simulink model "InductionHeating_bb_4"  (R2026b)
settings: Solver=FixedStepDiscrete  StopTime=0.008
PostLoadFcn:
  | Ts = 1e-6;Ts_fpga=10e-9;   R=3; Capa=300e-9;L=100e-6;Pejo_factor=1;
InitFcn:
  | Ts = 1e-6;Ts_fpga=10e-9;   R=3; Capa=300e-9;L=100e-6;Pejo_factor=1;
undefined symbols (not defined in the file or in its folder): DiscIntNeverNeededParam, ee_sli_rtmsupport, gcbh, isSetWhenUndefinedState, MATESOCwDio
libraries: fl_lib x67, nesl_utility x40, hdlsllib x32, simulink x15, eeGeneralControl x9, ee_lib x3
(part 3 of 7)

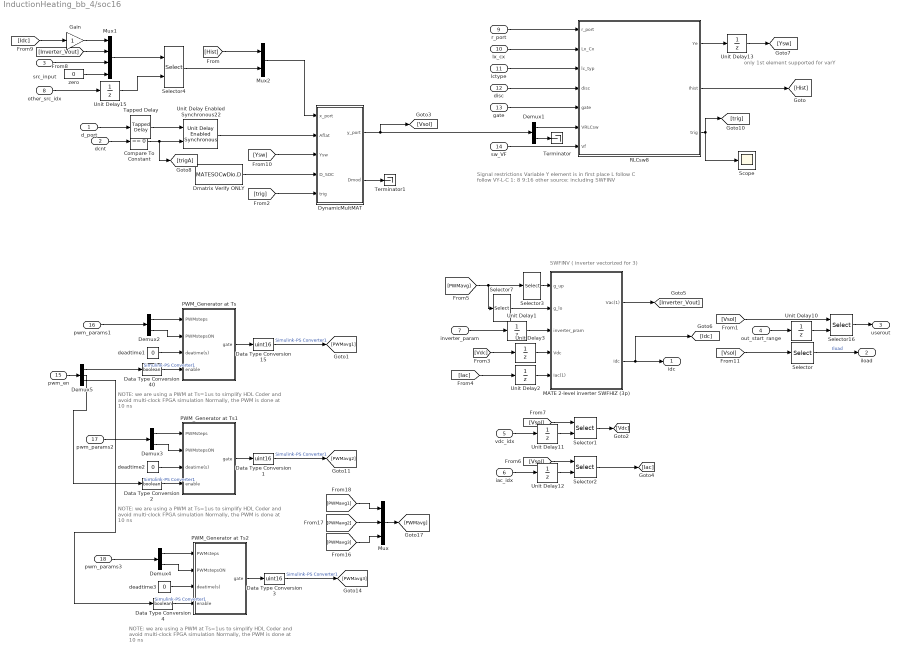
== system InductionHeating_bb_4/soc16 ==
  note: SWFINV ( inverter vectorized for 3)
  note: only 1st element supported for varY
  note: NOTE: we are using a PWM at Ts=1us to simplify HDL Coder
      | and avoid multi-clock FPGA simulation
      | Normally, the PWM is done at 10 ns
  note: Signal restrictions
      | Variable Y element is in first place
      | L follow
      | C follow
      | VY-L-C 1: 8
      | 9:16 other source: including SWFINV
  note: NOTE: we are using a PWM at Ts=1us to simplify HDL Coder
      | and avoid multi-clock FPGA simulation
      | Normally, the PWM is done at 10 ns
  note: NOTE: we are using a PWM at Ts=1us to simplify HDL Coder
      | and avoid multi-clock FPGA simulation
      | Normally, the PWM is done at 10 ns
  d_port : Inport
  dcnt : Inport  Port=2
  src_input : Inport  Port=3
  out_start_range : Inport  Port=4
  vdc_idx : Inport  Port=5
  iac_idx : Inport  Port=6
  inverter_param : Inport  Port=7
  other_src_idx : Inport  Port=8
  r_port : Inport  Port=9
  lx_cx : Inport  Port=10
  lctype : Inport  Port=11
  disc : Inport  Port=12
  gate : Inport  Port=13
  sw_VF : Inport  Port=14
  pwm_en : Inport  Port=15
  pwm_params1 : Inport  Port=16
  pwm_params2 : Inport  Port=17
  pwm_params3 : Inport  Port=18
  Compare To Constant : hdlsllib/Logic and Bit Operations/Compare To Constant  relop===  const=0  OutDataTypeStr=boolean
  Data Type Conversion1 : DataTypeConversion  OutDataTypeStr=uint16  RndMeth=Nearest  SaturateOnIntegerOverflow=off
  Data Type Conversion15 : DataTypeConversion  OutDataTypeStr=uint16  RndMeth=Nearest  SaturateOnIntegerOverflow=off
  Data Type Conversion2 : DataTypeConversion  OutDataTypeStr=boolean  RndMeth=Nearest  SaturateOnIntegerOverflow=off
  Data Type Conversion3 : DataTypeConversion  OutDataTypeStr=uint16  RndMeth=Nearest  SaturateOnIntegerOverflow=off
  Data Type Conversion4 : DataTypeConversion  OutDataTypeStr=boolean  RndMeth=Nearest  SaturateOnIntegerOverflow=off
  Data Type Conversion40 : DataTypeConversion  OutDataTypeStr=boolean  RndMeth=Nearest  SaturateOnIntegerOverflow=off
  Demux1 : Demux  Outputs=[8 8]
  Demux2 : Demux  Outputs=2
  Demux3 : Demux  Outputs=2
  Demux4 : Demux  Outputs=2
  Demux5 : Demux  Outputs=3
  Dmatrix Verify ONLY : Constant  Value=MATESOCwDio.D  OutDataTypeStr=single  SampleTime=Ts
  DynamicMultMAT : Subsystem
  Gain : Gain
  MATE 2-level inverter SWFHIZ (3p) : Subsystem  AncestorBlock=simetranss/FPGA/MATE 2-level inverter SWFHIZ (3ph)  mask(MATE Inverter Switching Function (2-level IGBT/Diode) (3-phase)){Ron=1e-3, Gpp=100, Gip=1e-6, Ts=Ts, min_charge=5}
      mask prompts: Ron "Switch Ron (Ohms)"; Gpp "Snubber resistance (Ohms)"; Gip "Snubber Capacitor (Ohms)"; Ts "Sample time (s)"; min_charge "Minimum rectifying current (A)"
      mask help:
      | This block implements a 3-phase  2-level inverter as a switching function.
      |
      | The block is Time-Step-Averaging-capable meaning that the averaging gate ON-time is averaged at each time step.
      |
      | With this approach, dead-times smaller than the sample time are accurately taken into account.
      |
      | The inverter can be in high impedance and rectifying states by selecting correctly the RC snubber.
      | Typically Rsnubber=L_load/Ts , then adjust Csnubber so Rsnubber*Csnubber=2*Ts.
      |
      | Minimum Rectifying current: In passive mode (no IGBT pulsing), this is the minimum rectifying current that is injected to the DC bus. This parameter is used to avoid unrealistic DC-bus charging when the inverter acts as a diode recfifier and do not impact in active control (gate pulsing) mode.
      |
      | The block has a constant admittance and is suitable for HDL coder.
  Mux : Mux  Inputs=3
  Mux1 : Mux  Inputs=[3 3 1 1]
  Mux2 : Mux  Inputs=[8 8]
  PWM_Generator at Ts : Subsystem
      mask Display: disp(' PWM \n Generator ')
  PWM_Generator at Ts1 : Subsystem
      mask Display: disp(' PWM \n Generator ')
  PWM_Generator at Ts2 : Subsystem
      mask Display: disp(' PWM \n Generator ')
  RLCsw8 : Subsystem  AncestorBlock=simetranss/FPGA/Variable discrete RLC  mask(Discrete variable High Accuracy Series RL or Parallel RC branch){typ=Pejovic Switch, discmeth=Backward Euler, Lon=1e-6, R=0, L=100e-6, Capa=300e-6, sbrl=on, Ts=Ts, showV=off, showI=off, Parameter11=|}
      mask Parameter11=|
      | bug list
      | Vf bug isw sign (27 08 2026)
      mask prompts: typ "Element type"; discmeth "Discretization"; Lon "Switch equivalent ON inductance (H)"; R "Initial Resistor resistance (Ohms)"; L "Initial Inductor inductance (H)"; Capa "Initial Capacitor capacitance (F)"; sbrl "Use signal-based RLC and parameter values"; Ts "Sample Time (s)"; showV "Show voltage port"; showI "Show current port"
      mask help:
      | This model implements a discretized  Series RL or Parallel RC branch that is on-line modifiable.
      |
      | On-line modifiable:  RLC parameters can be modified during simulation.
      |
      | Signals list (Vectors)
      |
      | R: resistance of either parallel RC or Series RL branch
      | Lx_Cx: inverse of capacitance (Parallel RC) or inductance (Series RL)
      | LC_type: 0 for Parallel RC, 1 for Series RL, 2 for Pejovic switch
      | disc: Choice of discretization method: 1 for Backward Euler (order 1) , 2 for Trapezoidal method (order 2), 3 for Radau IIA (5th order)
      |
      | gate: for chosen switches only, the corresponding gate signal (0 or 1)
      |
      | Use with R=0 (Series RL) to obtain a simple inductor.
      | Use with R=inf (Parallel RC) to obtain a simple capacitor.
      |
      | Note: Pejovic switches are always forced-simulated with Backward Eule with the inductance parameter value for ON state Lpejo=Ts and equivalent Open state capacitance Cpejo=Ts. Lpejo=Cpejo=Ts.
      mask init:
      | block=gcb; 
      | Xcomp=0;
      | s1=0;s2=0;s3=0;s4=0;r1=0;r2=0;l1=0;l2=0;
      | c1=0;c2=0;c3=0;c4=0;x1=0;x2=0;x3=0;x4=0;
      | 
      | MaskEnables =get_param (block ,'MaskEnables' ); 
      | discm=get_param(block,"discmeth");
      | if isequal(get_param(block,"discmeth"),'Backward Euler')
      |     dd=1;
      |     ddi=1;
      | elseif isequal(get_param(block,"discmeth"),'Trapezoidal')
      |     dd=2;
      |     ddi=2;
      | else
      |     dd=5;
      |     ddi=3;
      | end
      | sst=0;
      | br_typ=0;
      | is_sw=0;
      | 
      | % if isequal(get_param(block,"traprule"),'on')
      | %     Trapfactor=2;
      | % else
      | %     Trapfactor=1;
      | % end
      | RootMatch=0;
      | Ihist=0;
      | 
      | if isequal(get_param(block,"showV"),'on')
      |         replace_block (block ,'Followlinks' ,'on' ,'Name' ,'v' ,'BlockType' ,'Terminator' ,'Outport' ,'noprompt' ); 
      | else
      |         replace_block (block ,'Followlinks' ,'on' ,'Name' ,'v' ,'BlockType' ,'Outport' ,'Terminator' ,'noprompt' ); 
      | end
      | if isequal(get_param(block,"showI"),'on')
      |         replace_block (block ,'Followlinks' ,'on' ,'Name' ,'i' ,'BlockType' ,'Terminator' ,'Outport' ,'noprompt' ); 
      | else
      |         replace_block (block ,'Followlinks' ,'on' ,'Name' ,'i' ,'BlockType' ,'Outport' ,'Terminator' ,'noprompt' ); 
      | end
      | 
      | if isequal(get_param(block,"sbrl"),'on')
      |     replace_block (block ,'Followlinks' ,'on' ,'Name' ,'rlc' ,'BlockType' ,'Constant' ,'Inport' ,'noprompt' );
      |     MaskEnables {4 }='off' ;
      |     MaskEnables {5 }='off' ;
      |     MaskEnables {6 }='off' ;
      | else
      |     replace_block (block ,'Followlinks' ,'on' ,'Name' ,'rlc' ,'BlockType' ,'Inport' ,'Constant' ,'noprompt' );
      |     MaskEnables {4 }='on' ;
      |     MaskEnables {5 }='on' ;
      |     MaskEnables {6 }='on' ;
      | end
      | 
      | 
      | 
      | 
      | 
      | 
      | set_param (block ,'MaskEnables' ,MaskEnables ); 
      | qq='x';
      | 
      | typp=get_param(block,'typ');
      | % bp=get_param(block,'pcbp');
      | if isequal(typp,'Pejovic Switch')
      |     replace_block (block ,'Followlinks' ,'on' ,'Name' ,'gate' ,'BlockType' ,'Constant' ,'Inport' ,'noprompt' ); 
      |     %replace_block (block ,'Followlinks' ,'on' ,'Name' ,'init_in' ,'BlockType' ,'Inport' ,'Constant' ,'noprompt'  );
      |     %replace_block (block ,'Followlinks' ,'on' ,'Name' ,'init_out' ,'BlockType' ,'Outport' ,'Terminator' ,'noprompt'  );
      |     Rsw=Lon/Ts;
      |     txt='Switch';
      |     [s1,s2,s3,s4,r1,r2,l1,l2,c1,c2,c3,c4] = MATEdrawRLC('Series RLC Branch',0,1,0,'Open circuit');
      |     c2=[0 -20];
      |     c1=[30 120];
      |     qq='Switch';
      | % MaskEnables {2 }='on' ; 
      | % MaskEnables {3 }='off' ; 
      | % MaskEnables {4 }='off' ; 
      | % MaskEnables {5 }='off' ; 
      | % MaskEnables {6 }='off' ; 
      | % MaskEnables {8 }='off' ;
      | %force Backward Euler
      |     set_param(block,"discmeth",'Backward Euler')
      |     dd=1;
      |     ddi=1;
      |     is_sw=1;
      |     br_typ=0; % use Z=L/h 
      |  
      | elseif isequal(typp,'Inductor')
      |     replace_block (block ,'Followlinks' ,'on' ,'Name' ,'gate' ,'BlockType' ,'Inport' ,'Constant' ,'noprompt' ); 
      |     set_param([block '/gate'],'Value','1');
      |     replace_block (block ,'Followlinks' ,'on' ,'Name' ,'init_in' ,'BlockType' ,'Inport' ,'Constant' ,'noprompt'  ); 
      |     replace_block (block ,'Followlinks' ,'on' ,'Name' ,'init_out' ,'BlockType' ,'Outport' ,'Terminator' ,'noprompt'  );
      |  
      | 
      |     qq='Inductor';
      | % MaskEnables {2 }='off' ; 
      | % MaskEnables {3 }='on' ; 
      | % MaskEnables {4 }='off' ; 
      | % MaskEnables {5 }='on' ; 
      | % MaskEnables {6 }='off' ; 
      | % MaskEnables {8 }='off' ;
      |     x1=0;x2=0;x3=0;x4=0;
      |     if dd==5
      |         warning('Setting Inductor to Trapezoidal discretization');
      |         set_param(block,"discmeth",'Trapezoidal')
      |         dd=2;
      |     end
      |     [s1,s2,s3,s4,r1,r2,l1,l2,c1,c2,c3,c4] = MATEdrawRLC('Series RLC Branch',0,1,0,'L');
      |     [Ad,Bd1,Bd2,Cd,Dd,Y]=discRL(0,1/L,1,0,Ts,dd);
      |     Rsw=1/Y;
      | elseif isequal(typp,'Series RL')
      |     replace_block (block ,'Followlinks' ,'on' ,'Name' ,'gate' ,'BlockType' ,'Inport' ,'Constant' ,'noprompt' ); 
      |     set_param([block '/gate'],'Value','1');
      |     %replace_block (block ,'Followlinks' ,'on' ,'Name' ,'init_in' ,'BlockType' ,'Inport' ,'Constant' ,'noprompt'  ); 
      |     %replace_block (block ,'Followlinks' ,'on' ,'Name' ,'init_out' ,'BlockType' ,'Outport' ,'Terminator' ,'noprompt'  );
      | 
      |     [Ad,Bd1,Bd2,Cd,Dd,Y]=discRL(-R/L,1/L,1,0,Ts,dd);
      |     Rsw=1/Y;
      |     qq='Series RL';
      |     br_typ=0;
      |     sst=0;
      | % MaskEnables {2 }='off' ; 
      | % MaskEnables {3 }='on' ; 
      | % MaskEnables {4 }='off' ; 
      | if isequal(get_param(block,"sbrl"),'off')
      |   MaskEnables {4 }='on' ; 
      |   MaskEnables {5 }='on' ; 
      |   MaskEnables {6 }='off' ; 
      | end
      | % MaskEnables {8 }='off' ;
      |     x1=0;x2=0;x3=0;x4=0;
      |     [s1,s2,s3,s4,r1,r2,l1,l2,c1,c2,c3,c4] = MATEdrawRLC('Series RLC Branch',1,1,0,'RL');
      |     
      |     
      | elseif isequal(typp,'Parallel RC')
      |     replace_block (block ,'Followlinks' ,'on' ,'Name' ,'gate' ,'BlockType' ,'Inport' ,'Constant' ,'noprompt' ); 
      |     set_param([block '/gate'],'Value','0');
      |     %replace_block (block ,'Followlinks' ,'on' ,'Name' ,'init_in' ,'BlockType' ,'Inport' ,'Constant' ,'noprompt'  );
      |     %replace_block (block ,'Followlinks' ,'on' ,'Name' ,'init_out' ,'BlockType' ,'Outport' ,'Terminator' ,'noprompt'  );
      | if R<1e-6
      |     warndlg(['Resistance of RC block: ' block ' is very low for a Parallel RC Branch. Set R=inf if you really want an ideal capacitor with no parallel resistor.'],'MATE warning');
      | end
      |     qq='Capacitor';
      | % MaskEnables {2 }='off' ; 
      | % MaskEnables {3 }='off' ; 
      | % MaskEnables {4 }='on' ; 
      | if isequal(get_param(block,"sbrl"),'off')
      |   MaskEnables {4 }='on' ; 
      |   MaskEnables {5 }='off' ; 
      |   MaskEnables {6 }='on' ; 
      | end
      | 
      | % MaskEnables {8 }='off' ;
      |     % if dd==5 
      |     %     warning('Very low resistance. Setting Capacitor to Trapezoidal discretization');
      |     %     set_param(block,"discmeth",'Trapezoidal')
      |     %     dd=2;
      |     % end
      |     sst=1;
      |     br_typ=1;
      | 
      |     [Ad,Bd1,Bd2,Cd,Dd,Y]=discRL(-1/R/Capa,1/Capa,1,0,Ts,dd);
      |     Rsw=Y;
      | 
      |     if R>1e8
      |             [s1,s2,s3,s4,r1,r2,l1,l2,c1,c2,c3,c4,x1,x2,x3,x4] = MATEdrawRLC('Parallel RLC Branch',0,0,1,'C');
      |                 
      |     else
      |             [s1,s2,s3,s4,r1,r2,l1,l2,c1,c2,c3,c4,x1,x2,x3,x4] = MATEdrawRLC('Parallel RLC Branch',1,0,1,'RC');
      |                  s1=-20;s2=-120;s3=220;s4=120; %reframe
      | 
      |     end
      | 
      | 
      | elseif isequal(typp,'2-level inverter switch')
      |     replace_block (block ,'Followlinks' ,'on' ,'Name' ,'gate' ,'BlockType' ,'Constant' ,'Inport' ,'noprompt' ); 
      |     replace_block (block ,'Followlinks' ,'on' ,'Name' ,'init_in' ,'BlockType' ,'Constant' ,'Inport','noprompt'  );
      |     replace_block (block ,'Followlinks' ,'on' ,'Name' ,'init_out' ,'BlockType' ,'Terminator' ,'Outport' ,'noprompt'  );
      |     Rsw=Lon/Ts;
      |     txt='Inverter half';
      |     Xcomp=1;
      |     qq='Pejo Inverter Half';
      |     %force Backward Euler
      | set_param(block,'traprule','off');
      | % MaskEnables {2 }='on' ; 
      | % MaskEnables {3 }='off' ; 
      | % MaskEnables {4 }='off' ; 
      | % MaskEnables {5 }='off' ; 
      | % MaskEnables {6 }='off' ; 
      | % MaskEnables {8 }='on' ;
      |         [s1,s2,s3,s4,r1,r2,l1,l2,c1,c2,c3,c4] = MATEdrawRLC('Series RLC Branch',0,1,0,'Open circuit');
      |     c2=[0 -20];
      |     c1=[30 120];
      |         if dd==5  ||  dd==2
      |         set_param(block,"discmeth",'Backward Euler')
      |         dd=1;
      |         end
      | 
      | else
      | end
      | 
      | % if isequal(typp,'2-level inverter switch')  && isequal(bp,'on')
      | %         replace_block (block ,'Followlinks' ,'on' ,'Name' ,'Bypass' ,'BlockType' ,'Ground' ,'Inport' ,'noprompt' ); 
      | % else
      | %         replace_block (block ,'Followlinks' ,'on' ,'Name' ,'Bypass' ,'BlockType' ,'Inport' ,'Ground' ,'noprompt' ); 
      | % end
      | 
      | MaskEnables {7 }='on' ; 
      | set_param (block ,'MaskEnables' ,MaskEnables ); 
      | 
      | 
      | if Ts>2e-6
      |     %warndlg(['Sample Time of ' num2str(Ts) ' s. may be somehow large for the Pejovic switch to be accurate. Sample time below 2 us are recommended.'])
      | end
      | 
      | if isequal(get_param(block,"sbrl"),'on')
      |     x1=0;x2=0;x3=0;x4=0;
      |     [s1,s2,s3,s4,r1,r2,l1,l2,c1,c2,c3,c4] = MATEdrawRLC('Series RLC Branch',1,1,1,'RLC');
      | qq='External user choice';
      | 
      | end
      mask TypeOptions typ: Series RL | Parallel RC | Pejovic Switch
      mask TypeOptions discmeth: Backward Euler | Trapezoidal | Radau IIA 5th order
      mask DialogControl Control2 Prompt: The above RLC parameters will be used as default in SoC
      mask DialogControl Yvalue Prompt: tmp
      mask DialogControl Control4 Prompt: bugs
      mask DialogControl Control5 Prompt: Vf bug isw sign (27 08 2026)
      mask Display:
      | plot(s1,s2,s3,s4,r1,r2,l1,l2,c1,c2,c3,c4,x1,x2,x3,x4);
      | color('blue')
      | 
      | disp([qq  10 10])
  Scope : Scope
      settings: ActiveDisplayYMinimum=-0.06094  ActiveDisplayYMaximum=1.125  DataLoggingVariableName=ScopeData2
  Selector : Selector  InputPortWidth=16  IndexOptions=Index vector (dialog)  Indices=11  OutputSizes=1  RuntimeRangeChecks=off
  Selector1 : Selector  InputPortWidth=16  IndexOptions=Index vector (port)  Indices=[1:16]  OutputSizes=4  RuntimeRangeChecks=off
  Selector16 : Selector  InputPortWidth=16  IndexOptions=Starting index (port)  Indices=[1:16]  OutputSizes=5  RuntimeRangeChecks=off
  Selector2 : Selector  InputPortWidth=16  IndexOptions=Index vector (port)  Indices=[1:16]  OutputSizes=4  RuntimeRangeChecks=off
  Selector3 : Selector  InputPortWidth=6  IndexOptions=Index vector (dialog)  Indices=[1 3 5 ]  OutputSizes=1  RuntimeRangeChecks=off
  Selector4 : Selector  InputPortWidth=8  IndexOptions=Index vector (port)  Indices=[1:16]  OutputSizes=4  RuntimeRangeChecks=off
  Selector7 : Selector  InputPortWidth=6  IndexOptions=Index vector (dialog)  Indices=[1 3 5 ]+1  OutputSizes=1  RuntimeRangeChecks=off
  Tapped Delay : simulink/Discrete/Tapped Delay  vinit=0.0  samptime=-1  NumDelays=256  DelayOrder=Oldest  includeCurrent=off
      settings: LibrarySourceBlock=hdlsllib/Discrete/Tapped Delay
  Terminator : Terminator
  Terminator1 : Terminator
  Unit Delay Enabled Synchronous22 : hdlsllib/Discrete/Unit Delay Enabled Synchronous  InitialCondition=0.0  SampleTime=-1
  Unit Delay{1..3,13} (4 alike) : UnitDelay  SampleTime=Ts
  Unit Delay{10..12,15} (4 alike) : UnitDelay  InitialCondition=1  SampleTime=Ts
  deadtime1 : Constant  Value=0  SampleTime=Ts
  deadtime2 : Constant  Value=0  SampleTime=Ts
  deadtime3 : Constant  Value=0  SampleTime=Ts
  zero : Constant  Value=0  OutDataTypeStr=single  SampleTime=Ts
  idc : Outport
  iload : Outport  Port=2
  userout : Outport  Port=3
  wires:
  out_start_range/1 -> Unit Delay10/1
  Compare To Constant/1 -> [trigA], Unit Delay Enabled Synchronous22/2
  Tapped Delay/1 -> Unit Delay Enabled Synchronous22/1
  dcnt/1 -> Compare To Constant/1
  d_port/1 -> Tapped Delay/1
  [Hist] -> Mux2/1
  Unit Delay Enabled Synchronous22/1 -> DynamicMultMAT/2(Aflat)
  inverter_param/1 -> Unit Delay1/1
  Unit Delay2/1 -> MATE 2-level inverter SWFHIZ (3p)/5(Iac(1))
  [Vdc] -> Unit Delay3/1
  Unit Delay3/1 -> MATE 2-level inverter SWFHIZ (3p)/4(Vdc)
  MATE 2-level inverter SWFHIZ (3p)/2(Idc) -> [Idc], idc/1
  Selector1/1 -> [Vdc]
  [Vsol] -> Selector1/1
  [Vsol] -> Selector2/1
  Selector2/1 -> [Iac]
  [Idc] -> Gain/1
  [Inverter_Vout] -> Mux1/2
  src_input/1 -> Mux1/3
  Mux2/1 -> DynamicMultMAT/1(x_port)
  Mux1/1 -> Selector4/1
  [PWMavg] -> Selector7/1, Selector3/1
  deadtime1/1 -> PWM_Generator at Ts/3(deatime(s))
  Data Type Conversion40/1 -> PWM_Generator at Ts/4(enable)  "Simulink-PS Converter1"
  PWM_Generator at Ts/1(gate) -> Data Type Conversion15/1
  Dmatrix Verify ONLY/1 -> DynamicMultMAT/4(D_SOC)
  Demux1/1 -> RLCsw8/6(VRLCsw)
  Selector4/1 -> Mux2/2
  vdc_idx/1 -> Unit Delay11/1
  iac_idx/1 -> Unit Delay12/1
  other_src_idx/1 -> Unit Delay15/1
  zero/1 -> Mux1/4
  RLCsw8/3(trig) -> [trig], Scope/1
  RLCsw8/1(Ye) -> Unit Delay13/1
  [Ysw] -> DynamicMultMAT/3(Ysw)
  [trig] -> DynamicMultMAT/5(trig)
  MATE 2-level inverter SWFHIZ (3p)/1(Vac(1)) -> [Inverter_Vout]
  Demux1/2 -> Terminator/1
  RLCsw8/2(Ihist) -> [Hist]
  disc/1 -> RLCsw8/4(disc)
  lctype/1 -> RLCsw8/3(lc_typ)
  lx_cx/1 -> RLCsw8/2(Lx_Cx)
  r_port/1 -> RLCsw8/1(r_port)
  gate/1 -> RLCsw8/5(gate)
  Unit Delay10/1 -> Selector16/2
  pwm_params1/1 -> Demux2/1
  Unit Delay11/1 -> Selector1/2
  Unit Delay12/1 -> Selector2/2
  [Vsol] -> Selector/1
  [Vsol] -> Selector16/1
  Unit Delay15/1 -> Selector4/2
  Unit Delay13/1 -> [Ysw]
  Unit Delay1/1 -> MATE 2-level inverter SWFHIZ (3p)/3(inverter_pram)
  Data Type Conversion15/1 -> [PWMavg1]  "Simulink-PS Converter1"
  Selector/1 -> iload/1  "Iload"
  Selector3/1 -> MATE 2-level inverter SWFHIZ (3p)/1(g_up)
  Selector7/1 -> MATE 2-level inverter SWFHIZ (3p)/2(g_lo)
  Data Type Conversion1/1 -> [PWMavg2]  "Simulink-PS Converter1"
  pwm_params2/1 -> Demux3/1
  PWM_Generator at Ts1/1(gate) -> Data Type Conversion1/1
  Data Type Conversion2/1 -> PWM_Generator at Ts1/4(enable)  "Simulink-PS Converter1"
  deadtime2/1 -> PWM_Generator at Ts1/3(deatime(s))
  deadtime3/1 -> PWM_Generator at Ts2/3(deatime(s))
  Data Type Conversion4/1 -> PWM_Generator at Ts2/4(enable)  "Simulink-PS Converter1"
  PWM_Generator at Ts2/1(gate) -> Data Type Conversion3/1
  pwm_params3/1 -> Demux4/1
  Data Type Conversion3/1 -> [PWMavg3]  "Simulink-PS Converter1"
  pwm_en/1 -> Demux5/1
  Demux5/1 -> Data Type Conversion40/1
  Demux5/2 -> Data Type Conversion2/1
  Demux5/3 -> Data Type Conversion4/1
  [PWMavg2] -> Mux/2
  [PWMavg1] -> Mux/1
  [PWMavg3] -> Mux/3
  Mux/1 -> [PWMavg]
  Demux3/1 -> PWM_Generator at Ts1/1(PWMsteps)
  Demux3/2 -> PWM_Generator at Ts1/2(PWMstepsON)
  Demux4/1 -> PWM_Generator at Ts2/1(PWMsteps)
  Demux4/2 -> PWM_Generator at Ts2/2(PWMstepsON)
  Selector16/1 -> userout/1
  sw_VF/1 -> RLCsw8/7(Vf)
  Demux2/1 -> PWM_Generator at Ts/1(PWMsteps)
  Demux2/2 -> PWM_Generator at Ts/2(PWMstepsON)
  DynamicMultMAT/2(Dmod) -> Terminator1/1
  Gain/1 -> Mux1/1
  [Iac] -> Unit Delay2/1
  DynamicMultMAT/1(y_port) -> [Vsol], Demux1/1

== system InductionHeating_bb_4/Baseline Model running at 10 nanoseconds/Subsystem ==
  Current Sensor : fl_lib/Electrical/Electrical Sensors/Current Sensor
  PS-Simulink Converter : nesl_utility/PS-Simulink Converter  PhysicalDomain=network_engine_domain  SubClassName=ps_output  LeftPortType=input  RightPortType=output  PseudoPeriodic=off  Frequencies=[]  VectorFormat=1-D array  Unit=inherit  AffineConversion=off
  + : PMIOPort  Side=Left
  - : PMIOPort  Port=2  Side=Right
  i : Outport
  wires:
  PS-Simulink Converter/1 -> i/1
  connections:
  PS-Simulink Converter/LConn1 -- Current Sensor/RConn1
  Current Sensor/RConn2 -- -/RConn1
  +/RConn1 -- Current Sensor/LConn1

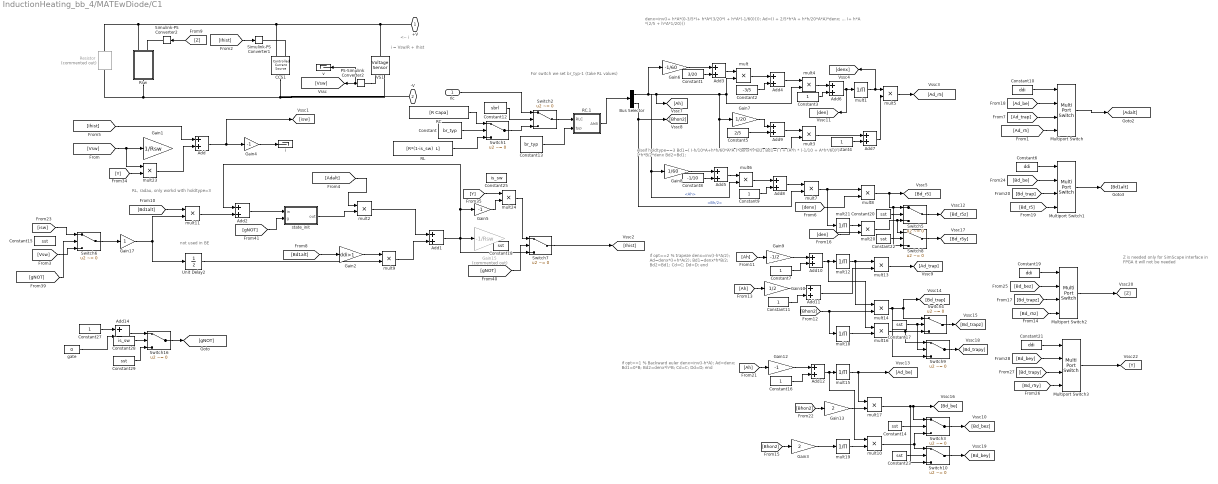
== system InductionHeating_bb_4/MATEwDiode/C1 ==
  note: not used in BE
  note: Z is needed only for SimScape interface
      | in FPGA it will not be needed
  note: i = Vsw/R + Ihist
  note: <-- i
  note: denx=inv(I+ h*A*(0-3/5*I+ h*A*(3/20*I + h*A*(-1/60))));
      | Ad=(I + 2/5*h*A + h*h/20*A*A)*denx;
      | ... I+ h*A *(2/5 + h*A*1/20)))
  note: elseif holdtype==3
      | Bd1=( I-h/10*A+h*h/60*A*A )*denx*h*B/2;
      | Bd1=( I + (A*h * (-1/10 + A*h*/60) ) )*h*B/2*denx
      | Bd2=Bd1;
  note: RL, radau, only workd with holdtype=3
  note: if opt==2 % trapeze
      | denx=inv(I-h*A/2);
      | Ad=denx*(I+h*A/2);
      | Bd1=denx*h*B/2;
      | Bd2=Bd1;
      | Cd=C;
      | Dd=D;
      | end
  note: if opt==1 % Backward euler
      | denx=inv(I-h*A);
      | Ad=denx;
      | Bd1=0*B;
      | Bd2=denx*h*B;
      | Cd=C;
      | Dd=D;
      | end
  note: For switch we set br_typ-1 (take RL values)
  rlc : Inport
  Add : Sum
  Add{1..12} (12 alike) : Sum  Inputs=2
  Add14 : Sum  Inputs=+-
  Bus Selector : BusSelector  OutputSignals=Ah,Bh/2
  CCS1 : fl_lib/Electrical/Electrical Sources/Controlled Current Source
  Constant : Constant  Value=br_typ
  Constant1 : Constant  Value=3/20  SampleTime=Ts
  Constant{6,10,19,21} (4 alike) : Constant  Value=ddi  SampleTime=Ts
  Constant{3..4,7,9,11,16,27} (7 alike) : Constant  SampleTime=Ts
  Constant12 : Constant  Value=sbrl
  Constant13 : Constant  Value=br_typ
  Constant{14..15,17..18,20,22..23,29} (8 alike) : Constant  Value=sst  SampleTime=Ts
  Constant2 : Constant  Value=-3/5  SampleTime=Ts
  Constant25 : Constant  Value=is_sw  SampleTime=Ts
  Constant28 : Constant  Value=is_sw  SampleTime=Ts
  Constant5 : Constant  Value=2/5  SampleTime=Ts
  Constant8 : Constant  Value=-1/10  SampleTime=Ts
  Gain1 : Gain  Gain=1/Rsw
  Gain10 : Gain  Gain=1/2
  Gain12 : Gain  Gain=-1
  Gain13 : Gain  Gain=2
  Gain15 : Gain  Commented=on  Gain=-1/Rsw
  Gain17 : Gain
  Gain2 : Gain  Gain=ddi>1
  Gain3 : Gain  Gain=2
  Gain4 : Gain  Gain=-1
  Gain5 : Gain  Gain=-1
  Gain6 : Gain  Gain=-1/60
  Gain7 : Gain  Gain=1/20
  Gain8 : Gain  Gain=1/60
  Gain9 : Gain  Gain=-1/2
  Multiport Switch{,1..3} (4 alike) : MultiPortSwitch  SaturateOnIntegerOverflow=off  InputSameDT=off
  PS-Simulink Converter2 : nesl_utility/PS-Simulink Converter  PhysicalDomain=network_engine_domain  SubClassName=ps_output  LeftPortType=input  RightPortType=output  PseudoPeriodic=off  Frequencies=[]  VectorFormat=inherit  Unit=inherit  AffineConversion=off
  RC : Constant  Value=[R Capa]  SampleTime=Ts
  RC.1 : Subsystem
  RL : Constant  Value="[R*(1-is_sw)  L]"  SampleTime=Ts
  Resistor : fl_lib/Electrical/Electrical Elements/Resistor  Commented=on  R=Rsw Ohm  i_specify=off  i_priority=None  i=0 A  i_nominal_specify=off  i_nominal_value=1  i_nominal_unit=A  v_specify=off  v_priority=None  v=0 V  v_nominal_specify=off  v_nominal_value=1  v_nominal_unit=V
  Rsw : Subsystem  mask(Simscape MATE variable resistance default value mask){defaultR=Rsw}
      mask prompts: defaultR "Default Resistance"
  Simulink-PS Converter1 : nesl_utility/Simulink-PS Converter  PhysicalDomain=network_engine_domain  SubClassName=ps_input  LeftPortType=input  RightPortType=output  PseudoPeriodic=off  Frequencies=[]  NoiseDistribution=none  NoiseParameters=[]  Unit=1  AffineConversion=off  FilteringAndDerivatives=provide  SimscapeFilterOrder=1  InputFilterTimeConstant=0.001  UdotUserProvided=0
  Simulink-PS Converter2 : nesl_utility/Simulink-PS Converter  PhysicalDomain=network_engine_domain  SubClassName=ps_input  LeftPortType=input  RightPortType=output  PseudoPeriodic=off  Frequencies=[]  NoiseDistribution=none  NoiseParameters=[]  Unit=1  AffineConversion=off  FilteringAndDerivatives=provide  SimscapeFilterOrder=1  InputFilterTimeConstant=0.001  UdotUserProvided=0
  Switch{1..10} (10 alike) : Switch  Criteria=u2 ~= 0  SaturateOnIntegerOverflow=off  InputSameDT=off
  Switch16 : Switch  Criteria=u2 ~= 0  Threshold=0.5  SaturateOnIntegerOverflow=off  InputSameDT=off
  Unit Delay2 : UnitDelay  SampleTime=-1
  VS1 : fl_lib/Electrical/Electrical Sensors/Voltage Sensor
  gate : Constant  Value=0
  i : Terminator
  mult{,2..11,13..14,16..17,20,23..24} (18 alike) : Product
  mult{1,12,15,18..19,21} (6 alike) : Product  Inputs=/
  state_init : Subsystem
  v : Terminator
  +V : PMIOPort  Side=Left
  -V : PMIOPort  Port=2  Side=Right
  wires:
  Switch7/1 -> [Ihist]
  gate/1 -> Add14/2
  mult20/1 -> Switch8/1, Switch5/3
  Constant20/1 -> Switch5/2
  Switch5/1 -> [Bd_r5z]
  mult21/1 -> mult20/1
  [den] -> mult20/2
  Switch3/1 -> [Bd_bez]
  Constant14/1 -> Switch3/2
  mult17/1 -> Switch10/3, [Bd_be], Switch3/1
  mult10/1 -> Switch10/1, Switch3/3
  mult19/1 -> mult10/2
  [Bhon2] -> Gain3/1
  Gain3/1 -> mult19/1
  mult18/1 -> mult16/2
  Constant13/1 -> RC.1/2(typ)
  RC.1/1(AhB) -> Bus Selector/1
  Constant12/1 -> Switch2/2
  rlc/1 -> Switch2/1
  Switch2/1 -> RC.1/1(RLC)
  Switch1/1 -> Switch2/3
  Constant/1 -> Switch1/2
  RL/1 -> Switch1/3
  RC/1 -> Switch1/1
  Gain2/1 -> mult9/1
  Constant10/1 -> Multiport Switch/1
  Constant6/1 -> Multiport Switch1/1
  Multiport Switch1/1 -> [Bd1alt]
  [Bd_be] -> Multiport Switch1/2
  [Bd_trap] -> Multiport Switch1/3
  [Bd_r5] -> Multiport Switch1/4
  Multiport Switch/1 -> [Adalt]
  [Ad_be] -> Multiport Switch/2
  [Ad_trap] -> Multiport Switch/3
  [Ad_r5] -> Multiport Switch/4
  Gain13/1 -> mult17/2
  [Ah] -> Gain12/1
  Gain12/1 -> Add12/1
  Constant16/1 -> Add12/2
  Add12/1 -> mult15/1, mult10/1
  [Bhon2] -> Gain13/1
  mult15/1 -> mult17/1, [Ad_be]
  mult11/1 -> Add2/2
  [Bd1alt] -> mult11/1
  [Bd1alt] -> Gain2/1
  mult9/1 -> Add1/2
  mult13/1 -> [Ad_trap]
  [Bhon2] -> mult14/2, mult18/1
  mult12/1 -> mult13/1, mult14/1
  [Ah] -> Gain10/1
  Gain10/1 -> Add11/1
  Constant11/1 -> Add11/2
  Add11/1 -> mult13/2
  Add10/1 -> mult12/1, mult16/1
  Constant7/1 -> Add10/2
  Gain9/1 -> Add10/1
  [Ah] -> Gain9/1
  [Z] -> Simulink-PS Converter2/1
  Bus Selector/2 -> [Bhon2], mult7/2  "<Bh/2>"
  Bus Selector/1 -> mult6/2, Gain8/1, mult/2, mult4/2, Gain7/1, mult3/2, [Ah], Gain6/1  "<Ah>"
  [denx] -> mult8/2
  mult7/1 -> mult8/1, mult21/1
  Add8/1 -> mult7/1
  Gain8/1 -> Add5/1
  Constant8/1 -> Add5/2
  mult6/1 -> Add8/1
  Add5/1 -> mult6/1
  Constant9/1 -> Add8/2
  mult5/1 -> [Ad_r5]
  mult1/1 -> mult5/1, [denx]
  [Adalt] -> mult2/1
  Add7/1 -> mult5/2
  mult3/1 -> Add7/1
  Gain7/1 -> Add9/1
  Add9/1 -> mult3/1
  Constant5/1 -> Add9/2
  Constant4/1 -> Add7/2
  Add6/1 -> mult1/1, [den]
  Constant3/1 -> Add6/2
  mult4/1 -> Add6/1
  Add4/1 -> mult4/1
  Constant2/1 -> Add4/2
  Add3/1 -> mult/1
  mult/1 -> Add4/1
  Constant1/1 -> Add3/2
  Gain6/1 -> Add3/1
  Unit Delay2/1 -> mult9/2
  Add1/1 -> Switch7/3, Gain5/1, Add2/1, Gain15/1
  Add2/1 -> state_init/1(in)
  Gain4/1 -> i/1
  [Ihist] -> Add/1
  PS-Simulink Converter2/1 -> [Vsw], v/1
  [Vsw] -> mult23/1, Gain1/1
  [Ihist] -> Simulink-PS Converter1/1
  Add/1 -> [isw], Gain4/1
  Switch6/1 -> Gain17/1
  [Vsw] -> Switch6/3
  [isw] -> Switch6/1
  mult2/1 -> Add1/1
  [Bd_r5z] -> Multiport Switch2/4
  [Bd_trapz] -> Multiport Switch2/3
  [Bd_bez] -> Multiport Switch2/2
  Multiport Switch2/1 -> [Z]
  Constant19/1 -> Multiport Switch2/1
  mult8/1 -> [Bd_r5], Switch8/3, Switch5/1
  Switch4/1 -> [Bd_trapz]
  Constant21/1 -> Multiport Switch3/1
  [Bd_bey] -> Multiport Switch3/2
  [Bd_trapy] -> Multiport Switch3/3
  [Bd_r5y] -> Multiport Switch3/4
  Switch8/1 -> [Bd_r5y]
  Constant22/1 -> Switch8/2
  Switch9/1 -> [Bd_trapy]
  Constant17/1 -> Switch9/2, Switch4/2
  mult16/1 -> Switch9/1, Switch4/3
  mult14/1 -> Switch9/3, [Bd_trap], Switch4/1
  Switch10/1 -> [Bd_bey]
  Constant23/1 -> Switch10/2
  Multiport Switch3/1 -> [Y]
  [Y] -> mult23/2
  mult23/1 -> Add/2
  mult24/1 -> Switch7/1
  [Y] -> mult24/1
  Gain5/1 -> mult24/2
  Gain17/1 -> mult11/2, Unit Delay2/1
  Constant27/1 -> Add14/1
  [gNOT] -> Switch6/2
  [gNOT] -> Switch7/2
  state_init/1(out) -> mult2/2
  [gNOT] -> state_init/2(g)
  Add14/1 -> Switch16/1
  Switch16/1 -> [gNOT]
  Constant28/1 -> Switch16/2
  Constant29/1 -> Switch16/3
  connections:
  Simulink-PS Converter2/RConn1 -- Rsw/LConn2
  Rsw/RConn1 -- Resistor/RConn1 -- VS1/RConn2 -- -V/RConn1 -- CCS1/LConn1
  PS-Simulink Converter2/LConn1 -- VS1/RConn1
  CCS1/RConn1 -- Simulink-PS Converter1/RConn1
  Rsw/LConn1 -- Resistor/LConn1 -- VS1/LConn1 -- +V/RConn1 -- CCS1/RConn2

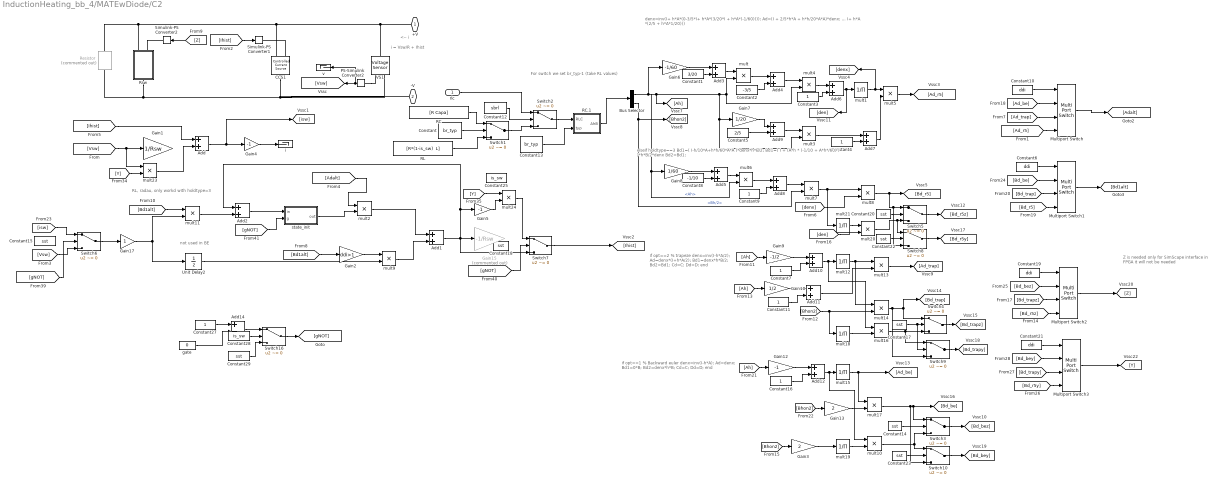
== system InductionHeating_bb_4/MATEwDiode/C2 ==
  note: not used in BE
  note: Z is needed only for SimScape interface
      | in FPGA it will not be needed
  note: i = Vsw/R + Ihist
  note: <-- i
  note: denx=inv(I+ h*A*(0-3/5*I+ h*A*(3/20*I + h*A*(-1/60))));
      | Ad=(I + 2/5*h*A + h*h/20*A*A)*denx;
      | ... I+ h*A *(2/5 + h*A*1/20)))
  note: elseif holdtype==3
      | Bd1=( I-h/10*A+h*h/60*A*A )*denx*h*B/2;
      | Bd1=( I + (A*h * (-1/10 + A*h*/60) ) )*h*B/2*denx
      | Bd2=Bd1;
  note: RL, radau, only workd with holdtype=3
  note: if opt==2 % trapeze
      | denx=inv(I-h*A/2);
      | Ad=denx*(I+h*A/2);
      | Bd1=denx*h*B/2;
      | Bd2=Bd1;
      | Cd=C;
      | Dd=D;
      | end
  note: if opt==1 % Backward euler
      | denx=inv(I-h*A);
      | Ad=denx;
      | Bd1=0*B;
      | Bd2=denx*h*B;
      | Cd=C;
      | Dd=D;
      | end
  note: For switch we set br_typ-1 (take RL values)
  rlc : Inport
  Add : Sum
  Add{1..12} (12 alike) : Sum  Inputs=2
  Add14 : Sum  Inputs=+-
  Bus Selector : BusSelector  OutputSignals=Ah,Bh/2
  CCS1 : fl_lib/Electrical/Electrical Sources/Controlled Current Source
  Constant : Constant  Value=br_typ
  Constant1 : Constant  Value=3/20  SampleTime=Ts
  Constant{6,10,19,21} (4 alike) : Constant  Value=ddi  SampleTime=Ts
  Constant{3..4,7,9,11,16,27} (7 alike) : Constant  SampleTime=Ts
  Constant12 : Constant  Value=sbrl
  Constant13 : Constant  Value=br_typ
  Constant{14..15,17..18,20,22..23,29} (8 alike) : Constant  Value=sst  SampleTime=Ts
  Constant2 : Constant  Value=-3/5  SampleTime=Ts
  Constant25 : Constant  Value=is_sw  SampleTime=Ts
  Constant28 : Constant  Value=is_sw  SampleTime=Ts
  Constant5 : Constant  Value=2/5  SampleTime=Ts
  Constant8 : Constant  Value=-1/10  SampleTime=Ts
  Gain1 : Gain  Gain=1/Rsw
  Gain10 : Gain  Gain=1/2
  Gain12 : Gain  Gain=-1
  Gain13 : Gain  Gain=2
  Gain15 : Gain  Commented=on  Gain=-1/Rsw
  Gain17 : Gain
  Gain2 : Gain  Gain=ddi>1
  Gain3 : Gain  Gain=2
  Gain4 : Gain  Gain=-1
  Gain5 : Gain  Gain=-1
  Gain6 : Gain  Gain=-1/60
  Gain7 : Gain  Gain=1/20
  Gain8 : Gain  Gain=1/60
  Gain9 : Gain  Gain=-1/2
  Multiport Switch{,1..3} (4 alike) : MultiPortSwitch  SaturateOnIntegerOverflow=off  InputSameDT=off
  PS-Simulink Converter2 : nesl_utility/PS-Simulink Converter  PhysicalDomain=network_engine_domain  SubClassName=ps_output  LeftPortType=input  RightPortType=output  PseudoPeriodic=off  Frequencies=[]  VectorFormat=inherit  Unit=inherit  AffineConversion=off
  RC : Constant  Value=[R Capa]  SampleTime=Ts
  RC.1 : Subsystem
  RL : Constant  Value="[R*(1-is_sw)  L]"  SampleTime=Ts
  Resistor : fl_lib/Electrical/Electrical Elements/Resistor  Commented=on  R=Rsw Ohm  i_specify=off  i_priority=None  i=0 A  i_nominal_specify=off  i_nominal_value=1  i_nominal_unit=A  v_specify=off  v_priority=None  v=0 V  v_nominal_specify=off  v_nominal_value=1  v_nominal_unit=V
  Rsw : Subsystem  mask(Simscape MATE variable resistance default value mask){defaultR=Rsw}
      mask prompts: defaultR "Default Resistance"
  Simulink-PS Converter1 : nesl_utility/Simulink-PS Converter  PhysicalDomain=network_engine_domain  SubClassName=ps_input  LeftPortType=input  RightPortType=output  PseudoPeriodic=off  Frequencies=[]  NoiseDistribution=none  NoiseParameters=[]  Unit=1  AffineConversion=off  FilteringAndDerivatives=provide  SimscapeFilterOrder=1  InputFilterTimeConstant=0.001  UdotUserProvided=0
  Simulink-PS Converter2 : nesl_utility/Simulink-PS Converter  PhysicalDomain=network_engine_domain  SubClassName=ps_input  LeftPortType=input  RightPortType=output  PseudoPeriodic=off  Frequencies=[]  NoiseDistribution=none  NoiseParameters=[]  Unit=1  AffineConversion=off  FilteringAndDerivatives=provide  SimscapeFilterOrder=1  InputFilterTimeConstant=0.001  UdotUserProvided=0
  Switch{1..10} (10 alike) : Switch  Criteria=u2 ~= 0  SaturateOnIntegerOverflow=off  InputSameDT=off
  Switch16 : Switch  Criteria=u2 ~= 0  Threshold=0.5  SaturateOnIntegerOverflow=off  InputSameDT=off
  Unit Delay2 : UnitDelay  SampleTime=-1
  VS1 : fl_lib/Electrical/Electrical Sensors/Voltage Sensor
  gate : Constant  Value=0
  i : Terminator
  mult{,2..11,13..14,16..17,20,23..24} (18 alike) : Product
  mult{1,12,15,18..19,21} (6 alike) : Product  Inputs=/
  state_init : Subsystem
  v : Terminator
  +V : PMIOPort  Side=Left
  -V : PMIOPort  Port=2  Side=Right
  wires:
  Switch7/1 -> [Ihist]
  gate/1 -> Add14/2
  mult20/1 -> Switch8/1, Switch5/3
  Constant20/1 -> Switch5/2
  Switch5/1 -> [Bd_r5z]
  mult21/1 -> mult20/1
  [den] -> mult20/2
  Switch3/1 -> [Bd_bez]
  Constant14/1 -> Switch3/2
  mult17/1 -> Switch10/3, [Bd_be], Switch3/1
  mult10/1 -> Switch10/1, Switch3/3
  mult19/1 -> mult10/2
  [Bhon2] -> Gain3/1
  Gain3/1 -> mult19/1
  mult18/1 -> mult16/2
  Constant13/1 -> RC.1/2(typ)
  RC.1/1(AhB) -> Bus Selector/1
  Constant12/1 -> Switch2/2
  rlc/1 -> Switch2/1
  Switch2/1 -> RC.1/1(RLC)
  Switch1/1 -> Switch2/3
  Constant/1 -> Switch1/2
  RL/1 -> Switch1/3
  RC/1 -> Switch1/1
  Gain2/1 -> mult9/1
  Constant10/1 -> Multiport Switch/1
  Constant6/1 -> Multiport Switch1/1
  Multiport Switch1/1 -> [Bd1alt]
  [Bd_be] -> Multiport Switch1/2
  [Bd_trap] -> Multiport Switch1/3
  [Bd_r5] -> Multiport Switch1/4
  Multiport Switch/1 -> [Adalt]
  [Ad_be] -> Multiport Switch/2
  [Ad_trap] -> Multiport Switch/3
  [Ad_r5] -> Multiport Switch/4
  Gain13/1 -> mult17/2
  [Ah] -> Gain12/1
  Gain12/1 -> Add12/1
  Constant16/1 -> Add12/2
  Add12/1 -> mult15/1, mult10/1
  [Bhon2] -> Gain13/1
  mult15/1 -> mult17/1, [Ad_be]
  mult11/1 -> Add2/2
  [Bd1alt] -> mult11/1
  [Bd1alt] -> Gain2/1
  mult9/1 -> Add1/2
  mult13/1 -> [Ad_trap]
  [Bhon2] -> mult14/2, mult18/1
  mult12/1 -> mult13/1, mult14/1
  [Ah] -> Gain10/1
  Gain10/1 -> Add11/1
  Constant11/1 -> Add11/2
  Add11/1 -> mult13/2
  Add10/1 -> mult12/1, mult16/1
  Constant7/1 -> Add10/2
  Gain9/1 -> Add10/1
  [Ah] -> Gain9/1
  [Z] -> Simulink-PS Converter2/1
  Bus Selector/2 -> [Bhon2], mult7/2  "<Bh/2>"
  Bus Selector/1 -> mult6/2, Gain8/1, mult/2, mult4/2, Gain7/1, mult3/2, [Ah], Gain6/1  "<Ah>"
  [denx] -> mult8/2
  mult7/1 -> mult8/1, mult21/1
  Add8/1 -> mult7/1
  Gain8/1 -> Add5/1
  Constant8/1 -> Add5/2
  mult6/1 -> Add8/1
  Add5/1 -> mult6/1
  Constant9/1 -> Add8/2
  mult5/1 -> [Ad_r5]
  mult1/1 -> mult5/1, [denx]
  [Adalt] -> mult2/1
  Add7/1 -> mult5/2
  mult3/1 -> Add7/1
  Gain7/1 -> Add9/1
  Add9/1 -> mult3/1
  Constant5/1 -> Add9/2
  Constant4/1 -> Add7/2
  Add6/1 -> mult1/1, [den]
  Constant3/1 -> Add6/2
  mult4/1 -> Add6/1
  Add4/1 -> mult4/1
  Constant2/1 -> Add4/2
  Add3/1 -> mult/1
  mult/1 -> Add4/1
  Constant1/1 -> Add3/2
  Gain6/1 -> Add3/1
  Unit Delay2/1 -> mult9/2
  Add1/1 -> Switch7/3, Gain5/1, Add2/1, Gain15/1
  Add2/1 -> state_init/1(in)
  Gain4/1 -> i/1
  [Ihist] -> Add/1
  PS-Simulink Converter2/1 -> [Vsw], v/1
  [Vsw] -> mult23/1, Gain1/1
  [Ihist] -> Simulink-PS Converter1/1
  Add/1 -> [isw], Gain4/1
  Switch6/1 -> Gain17/1
  [Vsw] -> Switch6/3
  [isw] -> Switch6/1
  mult2/1 -> Add1/1
  [Bd_r5z] -> Multiport Switch2/4
  [Bd_trapz] -> Multiport Switch2/3
  [Bd_bez] -> Multiport Switch2/2
  Multiport Switch2/1 -> [Z]
  Constant19/1 -> Multiport Switch2/1
  mult8/1 -> [Bd_r5], Switch8/3, Switch5/1
  Switch4/1 -> [Bd_trapz]
  Constant21/1 -> Multiport Switch3/1
  [Bd_bey] -> Multiport Switch3/2
  [Bd_trapy] -> Multiport Switch3/3
  [Bd_r5y] -> Multiport Switch3/4
  Switch8/1 -> [Bd_r5y]
  Constant22/1 -> Switch8/2
  Switch9/1 -> [Bd_trapy]
  Constant17/1 -> Switch9/2, Switch4/2
  mult16/1 -> Switch9/1, Switch4/3
  mult14/1 -> Switch9/3, [Bd_trap], Switch4/1
  Switch10/1 -> [Bd_bey]
  Constant23/1 -> Switch10/2
  Multiport Switch3/1 -> [Y]
  [Y] -> mult23/2
  mult23/1 -> Add/2
  mult24/1 -> Switch7/1
  [Y] -> mult24/1
  Gain5/1 -> mult24/2
  Gain17/1 -> mult11/2, Unit Delay2/1
  Constant27/1 -> Add14/1
  [gNOT] -> Switch6/2
  [gNOT] -> Switch7/2
  state_init/1(out) -> mult2/2
  [gNOT] -> state_init/2(g)
  Add14/1 -> Switch16/1
  Switch16/1 -> [gNOT]
  Constant28/1 -> Switch16/2
  Constant29/1 -> Switch16/3
  connections:
  Simulink-PS Converter2/RConn1 -- Rsw/LConn2
  Rsw/RConn1 -- Resistor/RConn1 -- VS1/RConn2 -- -V/RConn1 -- CCS1/LConn1
  PS-Simulink Converter2/LConn1 -- VS1/RConn1
  CCS1/RConn1 -- Simulink-PS Converter1/RConn1
  Rsw/LConn1 -- Resistor/LConn1 -- VS1/LConn1 -- +V/RConn1 -- CCS1/RConn2

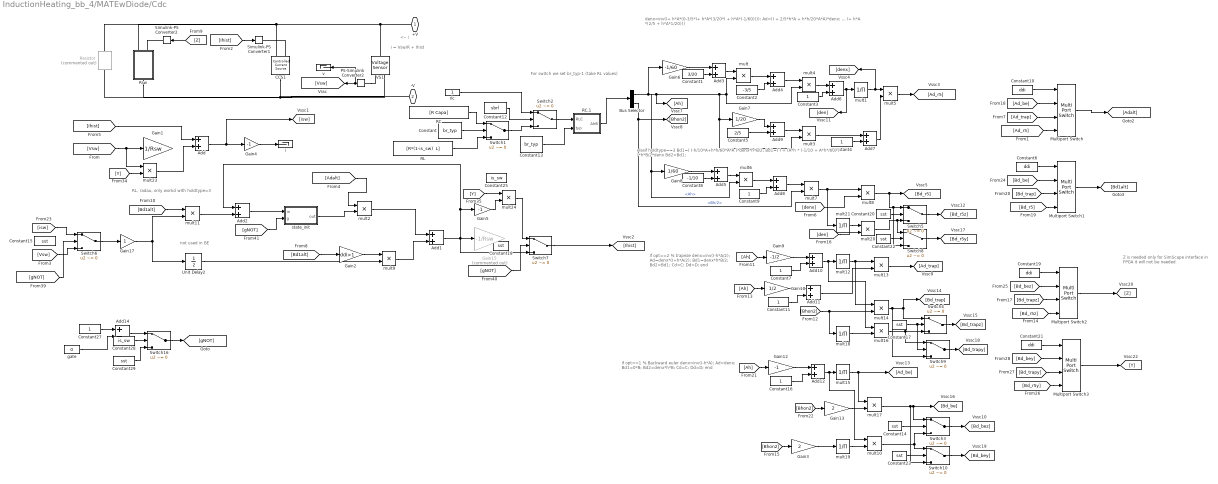
== system InductionHeating_bb_4/MATEwDiode/Cdc ==
  note: For switch we set br_typ-1 (take RL values)
  note: if opt==1 % Backward euler
      | denx=inv(I-h*A);
      | Ad=denx;
      | Bd1=0*B;
      | Bd2=denx*h*B;
      | Cd=C;
      | Dd=D;
      | end
  note: if opt==2 % trapeze
      | denx=inv(I-h*A/2);
      | Ad=denx*(I+h*A/2);
      | Bd1=denx*h*B/2;
      | Bd2=Bd1;
      | Cd=C;
      | Dd=D;
      | end
  note: RL, radau, only workd with holdtype=3
  note: elseif holdtype==3
      | Bd1=( I-h/10*A+h*h/60*A*A )*denx*h*B/2;
      | Bd1=( I + (A*h * (-1/10 + A*h*/60) ) )*h*B/2*denx
      | Bd2=Bd1;
  note: denx=inv(I+ h*A*(0-3/5*I+ h*A*(3/20*I + h*A*(-1/60))));
      | Ad=(I + 2/5*h*A + h*h/20*A*A)*denx;
      | ... I+ h*A *(2/5 + h*A*1/20)))
  note: <-- i
  note: i = Vsw/R + Ihist
  note: Z is needed only for SimScape interface
      | in FPGA it will not be needed
  note: not used in BE
  Add : Sum
  Add{1..12} (12 alike) : Sum  Inputs=2
  Add14 : Sum  Inputs=+-
  Bus Selector : BusSelector  OutputSignals=Ah,Bh/2
  CCS1 : fl_lib/Electrical/Electrical Sources/Controlled Current Source
  Constant : Constant  Value=br_typ
  Constant1 : Constant  Value=3/20  SampleTime=Ts
  Constant{6,10,19,21} (4 alike) : Constant  Value=ddi  SampleTime=Ts
  Constant{3..4,7,9,11,16,27} (7 alike) : Constant  SampleTime=Ts
  Constant12 : Constant  Value=sbrl
  Constant13 : Constant  Value=br_typ
  Constant{14..15,17..18,20,22..23,29} (8 alike) : Constant  Value=sst  SampleTime=Ts
  Constant2 : Constant  Value=-3/5  SampleTime=Ts
  Constant25 : Constant  Value=is_sw  SampleTime=Ts
  Constant28 : Constant  Value=is_sw  SampleTime=Ts
  Constant5 : Constant  Value=2/5  SampleTime=Ts
  Constant8 : Constant  Value=-1/10  SampleTime=Ts
  Gain1 : Gain  Gain=1/Rsw
  Gain10 : Gain  Gain=1/2
  Gain12 : Gain  Gain=-1
  Gain13 : Gain  Gain=2
  Gain15 : Gain  Commented=on  Gain=-1/Rsw
  Gain17 : Gain
  Gain2 : Gain  Gain=ddi>1
  Gain3 : Gain  Gain=2
  Gain4 : Gain  Gain=-1
  Gain5 : Gain  Gain=-1
  Gain6 : Gain  Gain=-1/60
  Gain7 : Gain  Gain=1/20
  Gain8 : Gain  Gain=1/60
  Gain9 : Gain  Gain=-1/2
  Multiport Switch{,1..3} (4 alike) : MultiPortSwitch  SaturateOnIntegerOverflow=off  InputSameDT=off
  PS-Simulink Converter2 : nesl_utility/PS-Simulink Converter  PhysicalDomain=network_engine_domain  SubClassName=ps_output  LeftPortType=input  RightPortType=output  PseudoPeriodic=off  Frequencies=[]  VectorFormat=inherit  Unit=inherit  AffineConversion=off
  RC : Constant  Value=[R Capa]  SampleTime=Ts
  RC.1 : Subsystem
  RL : Constant  Value="[R*(1-is_sw)  L]"  SampleTime=Ts
  Resistor : fl_lib/Electrical/Electrical Elements/Resistor  Commented=on  R=Rsw Ohm  i_specify=off  i_priority=None  i=0 A  i_nominal_specify=off  i_nominal_value=1  i_nominal_unit=A  v_specify=off  v_priority=None  v=0 V  v_nominal_specify=off  v_nominal_value=1  v_nominal_unit=V
  Rsw : Subsystem  mask(Simscape MATE variable resistance default value mask){defaultR=Rsw}
      mask prompts: defaultR "Default Resistance"
  Simulink-PS Converter1 : nesl_utility/Simulink-PS Converter  PhysicalDomain=network_engine_domain  SubClassName=ps_input  LeftPortType=input  RightPortType=output  PseudoPeriodic=off  Frequencies=[]  NoiseDistribution=none  NoiseParameters=[]  Unit=1  AffineConversion=off  FilteringAndDerivatives=provide  SimscapeFilterOrder=1  InputFilterTimeConstant=0.001  UdotUserProvided=0
  Simulink-PS Converter2 : nesl_utility/Simulink-PS Converter  PhysicalDomain=network_engine_domain  SubClassName=ps_input  LeftPortType=input  RightPortType=output  PseudoPeriodic=off  Frequencies=[]  NoiseDistribution=none  NoiseParameters=[]  Unit=1  AffineConversion=off  FilteringAndDerivatives=provide  SimscapeFilterOrder=1  InputFilterTimeConstant=0.001  UdotUserProvided=0
  Switch{1..10} (10 alike) : Switch  Criteria=u2 ~= 0  SaturateOnIntegerOverflow=off  InputSameDT=off
  Switch16 : Switch  Criteria=u2 ~= 0  Threshold=0.5  SaturateOnIntegerOverflow=off  InputSameDT=off
  Unit Delay2 : UnitDelay  SampleTime=-1
  VS1 : fl_lib/Electrical/Electrical Sensors/Voltage Sensor
  gate : Constant  Value=0
  i : Terminator
  mult{,2..11,13..14,16..17,20,23..24} (18 alike) : Product
  mult{1,12,15,18..19,21} (6 alike) : Product  Inputs=/
  rlc : Constant
  state_init : Subsystem
  v : Terminator
  +V : PMIOPort  Side=Left
  -V : PMIOPort  Port=2  Side=Right
  wires:
  Constant29/1 -> Switch16/3
  Constant28/1 -> Switch16/2
  Switch16/1 -> [gNOT]
  Add14/1 -> Switch16/1
  [gNOT] -> state_init/2(g)
  state_init/1(out) -> mult2/2
  [gNOT] -> Switch7/2
  [gNOT] -> Switch6/2
  Constant27/1 -> Add14/1
  Gain17/1 -> Unit Delay2/1, mult11/2
  Gain5/1 -> mult24/2
  [Y] -> mult24/1
  mult24/1 -> Switch7/1
  mult23/1 -> Add/2
  [Y] -> mult23/2
  Multiport Switch3/1 -> [Y]
  Constant23/1 -> Switch10/2
  Switch10/1 -> [Bd_bey]
  mult14/1 -> Switch4/1, [Bd_trap], Switch9/3
  mult16/1 -> Switch4/3, Switch9/1
  Constant17/1 -> Switch4/2, Switch9/2
  Switch9/1 -> [Bd_trapy]
  Constant22/1 -> Switch8/2
  Switch8/1 -> [Bd_r5y]
  [Bd_r5y] -> Multiport Switch3/4
  [Bd_trapy] -> Multiport Switch3/3
  [Bd_bey] -> Multiport Switch3/2
  Constant21/1 -> Multiport Switch3/1
  Switch4/1 -> [Bd_trapz]
  mult8/1 -> Switch5/1, Switch8/3, [Bd_r5]
  Constant19/1 -> Multiport Switch2/1
  Multiport Switch2/1 -> [Z]
  [Bd_bez] -> Multiport Switch2/2
  [Bd_trapz] -> Multiport Switch2/3
  [Bd_r5z] -> Multiport Switch2/4
  mult2/1 -> Add1/1
  [isw] -> Switch6/1
  [Vsw] -> Switch6/3
  Switch6/1 -> Gain17/1
  Add/1 -> Gain4/1, [isw]
  [Ihist] -> Simulink-PS Converter1/1
  [Vsw] -> Gain1/1, mult23/1
  PS-Simulink Converter2/1 -> v/1, [Vsw]
  [Ihist] -> Add/1
  Gain4/1 -> i/1
  Add2/1 -> state_init/1(in)
  Add1/1 -> Gain15/1, Add2/1, Gain5/1, Switch7/3
  Unit Delay2/1 -> mult9/2
  Gain6/1 -> Add3/1
  Constant1/1 -> Add3/2
  mult/1 -> Add4/1
  Add3/1 -> mult/1
  Constant2/1 -> Add4/2
  Add4/1 -> mult4/1
  mult4/1 -> Add6/1
  Constant3/1 -> Add6/2
  Add6/1 -> [den], mult1/1
  Constant4/1 -> Add7/2
  Constant5/1 -> Add9/2
  Add9/1 -> mult3/1
  Gain7/1 -> Add9/1
  mult3/1 -> Add7/1
  Add7/1 -> mult5/2
  [Adalt] -> mult2/1
  mult1/1 -> [denx], mult5/1
  mult5/1 -> [Ad_r5]
  Constant9/1 -> Add8/2
  Add5/1 -> mult6/1
  mult6/1 -> Add8/1
  Constant8/1 -> Add5/2
  Gain8/1 -> Add5/1
  Add8/1 -> mult7/1
  mult7/1 -> mult21/1, mult8/1
  [denx] -> mult8/2
  Bus Selector/1 -> Gain6/1, [Ah], mult3/2, Gain7/1, mult4/2, mult/2, Gain8/1, mult6/2  "<Ah>"
  Bus Selector/2 -> mult7/2, [Bhon2]  "<Bh/2>"
  [Z] -> Simulink-PS Converter2/1
  [Ah] -> Gain9/1
  Gain9/1 -> Add10/1
  Constant7/1 -> Add10/2
  Add10/1 -> mult16/1, mult12/1
  Add11/1 -> mult13/2
  Constant11/1 -> Add11/2
  Gain10/1 -> Add11/1
  [Ah] -> Gain10/1
  mult12/1 -> mult14/1, mult13/1
  [Bhon2] -> mult18/1, mult14/2
  mult13/1 -> [Ad_trap]
  mult9/1 -> Add1/2
  [Bd1alt] -> Gain2/1
  [Bd1alt] -> mult11/1
  mult11/1 -> Add2/2
  mult15/1 -> [Ad_be], mult17/1
  [Bhon2] -> Gain13/1
  Add12/1 -> mult10/1, mult15/1
  Constant16/1 -> Add12/2
  Gain12/1 -> Add12/1
  [Ah] -> Gain12/1
  Gain13/1 -> mult17/2
  [Ad_r5] -> Multiport Switch/4
  [Ad_trap] -> Multiport Switch/3
  [Ad_be] -> Multiport Switch/2
  Multiport Switch/1 -> [Adalt]
  [Bd_r5] -> Multiport Switch1/4
  [Bd_trap] -> Multiport Switch1/3
  [Bd_be] -> Multiport Switch1/2
  Multiport Switch1/1 -> [Bd1alt]
  Constant6/1 -> Multiport Switch1/1
  Constant10/1 -> Multiport Switch/1
  Gain2/1 -> mult9/1
  RC/1 -> Switch1/1
  RL/1 -> Switch1/3
  Constant/1 -> Switch1/2
  Switch1/1 -> Switch2/3
  Switch2/1 -> RC.1/1(RLC)
  rlc/1 -> Switch2/1
  Constant12/1 -> Switch2/2
  RC.1/1(AhB) -> Bus Selector/1
  Constant13/1 -> RC.1/2(typ)
  mult18/1 -> mult16/2
  Gain3/1 -> mult19/1
  [Bhon2] -> Gain3/1
  mult19/1 -> mult10/2
  mult10/1 -> Switch3/3, Switch10/1
  mult17/1 -> Switch3/1, [Bd_be], Switch10/3
  Constant14/1 -> Switch3/2
  Switch3/1 -> [Bd_bez]
  [den] -> mult20/2
  mult21/1 -> mult20/1
  Switch5/1 -> [Bd_r5z]
  Constant20/1 -> Switch5/2
  mult20/1 -> Switch5/3, Switch8/1
  gate/1 -> Add14/2
  Switch7/1 -> [Ihist]
  connections:
  CCS1/RConn2 -- +V/RConn1 -- VS1/LConn1 -- Resistor/LConn1 -- Rsw/LConn1
  CCS1/RConn1 -- Simulink-PS Converter1/RConn1
  PS-Simulink Converter2/LConn1 -- VS1/RConn1
  CCS1/LConn1 -- -V/RConn1 -- VS1/RConn2 -- Resistor/RConn1 -- Rsw/RConn1
  Simulink-PS Converter2/RConn1 -- Rsw/LConn2
